simulink model "ATOM_parking_chain"  (R2026a)
settings: Solver=ode4  StopTime=100  FixedStep=0.01
StopFcn:
  | % Put every new figure in the same MATLAB Figures window as a docked tab.
  | set(groot, 'defaultFigureWindowStyle', 'docked');
  | 
  | if exist('costmap_active', 'var') && ...
  |         exist('vehicle', 'var') && ...
  |         exist('parking_path', 'var') && ...
  |         ~isempty(parking_path)
  | 
  |     plotPlan(costmap_active, vehicle, parking_path);
  | 
  | else
  | 
  |     warning('No valid parking path is available for plotting.');
  | 
  | end
  | 
  | PlotControllerReferences( ...
  |     out.controller_reference_log);
  | 
  | PlotControllerTracking( ...
  |     out.controller_tracking_log);
undefined symbols (not defined in the file): lateral, longitudinal, stanley, vehicle
(part 10 of 11)

== matlab function ATOM_parking_chain/Plot vehicle1/Plot Vehicle Rear reference frame ==
  settings: updateMethod=DISCRETE
  data: kinematic input Bus: KinematicStateBus; steer_front input double; steer_rear input double; veh input; traj input; costmap input
   function plotVehicleRear(kinematic, steer_front, steer_rear, veh, traj, costmap)
  coder.extrinsic('imagesc','colormap','evalin');
%% Vehicle parameters

L  = veh(3);
track = veh(4);

front_overhang = veh(5);
rear_overhang  = veh(6);
left_overhang = veh(7);
right_overhang = veh(8);

vehicle_length  = L + front_overhang + rear_overhang;
vehicle_width = track + left_overhang + right_overhang;

wheel_width = veh(2);
wheel_radius = veh(1);

%% Reference trajectory

x_ref = evalin('base', 'parking_path(:,1)');
y_ref = evalin('base', 'parking_path(:,2)');


%% Current kinematic state

x = kinematic.pose.position.x;
y = kinematic.pose.position.y;

qz = kinematic.pose.orientation.z;
qw = kinematic.pose.orientation.w;

yaw = 2*atan2(qz,qw);

vx = kinematic.twist.linear.x;

steer_front = steer_front;
steer_rear = steer_rear;

%% Position and orientation vehicle body

vehicle_body = [L+front_overhang vehicle_width/2;
                L+front_overhang -vehicle_width/2;
                -rear_overhang -vehicle_width/2;
                -rear_overhang vehicle_width/2;
                L+front_overhang vehicle_width/2];

R_body = [ cos(yaw) -sin(yaw)
    sin(yaw)  cos(yaw) ];

body_world = (R_body*vehicle_body')';

body_world(:,1)=body_world(:,1)+x;
body_world(:,2)=body_world(:,2)+y;


%% Position and orientation wheels

wheel_body = [wheel_radius  wheel_width/2
                wheel_radius -wheel_width/2
                -wheel_radius -wheel_width/2
                -wheel_radius  wheel_width/2
                wheel_radius  wheel_width/2];

FL = [L  track/2];
FR = [L -track/2];
RL = [0  track/2];
RR = [0 -track/2];

centers = [FL;
    FR;
    RL;
    RR];

centers = (R_body*centers')';

centers(:,1) = centers(:,1)+x;
centers(:,2) = centers(:,2)+y;

wheelFL = transformWheel(centers(1,:),steer_front,yaw,wheel_body);
wheelFR = transformWheel(centers(2,:),steer_front,yaw,wheel_body);
wheelRL = transformWheel(centers(3,:),steer_rear,yaw,wheel_body);
wheelRR = transformWheel(centers(4,:),steer_rear,yaw,wheel_body);



persistent hFig
persistent ax
persistent hBody
persistent hWheelFL
persistent hWheelFR
persistent hWheelRL
persistent hWheelRR
persistent hTrajectory
persistent TrajX
persistent TrajY
persistent hRefTraj 


if isempty(hBody)
    hFig = figure(20);
    clf

    ax = axes(hFig);

    hold(ax,'on')
    axis(ax,'equal')
    grid(ax,'on')


    xlabel(ax,'x [m]')
    ylabel(ax,'y [m]')

    % --- obstacles: the same costmap the planner used ---
    res = double(costmap.info.resolution);
    W   = double(costmap.info.width);
    H   = double(costmap.info.height);
    ox  = double(costmap.info.origin.position.x);
    oy  = double(costmap.info.origin.position.y);
    g   = double(costmap.data);
    imagesc(ax, ox+(0:W-1)*res, oy+(0:H-1)*res, g, 'AlphaData', (g>=100)*0.55);
    colormap(ax, [1 1 1; 0.85 0.25 0.25]);
    set(ax, 'YDir','normal', 'Layer','top');

    hBody = plot(body_world(:,1),...
        body_world(:,2),...
        'k','LineWidth',2);

    hWheelFL = plot(wheelFL(:,1),...
        wheelFL(:,2),...
        'r','LineWidth',2);

    hWheelFR = plot(wheelFR(:,1),...
        wheelFR(:,2),...
        'r','LineWidth',2);

    hWheelRL = plot(wheelRL(:,1),...
        wheelRL(:,2),...
        'b','LineWidth',2);

    hWheelRR = plot(wheelRR(:,1),...
        wheelRR(:,2),...
        'b','LineWidth',2);

    TrajX = x;
    TrajY = y;

   hTrajectory = plot(TrajX, TrajY, 'g', 'LineWidth', 3);
   hRefTraj    = plot(x_ref, y_ref, 'b', 'LineWidth', 1);

else

    set(hBody,...
        'XData',body_world(:,1),...
        'YData',body_world(:,2));

    set(hWheelFL,...
        'XData',wheelFL(:,1),...
        'YData',wheelFL(:,2));

    set(hWheelFR,...
        'XData',wheelFR(:,1),...
        'YData',wheelFR(:,2));

    set(hWheelRL,...
        'XData',wheelRL(:,1),...
        'YData',wheelRL(:,2));

    set(hWheelRR,...
        'XData',wheelRR(:,1),...
        'YData',wheelRR(:,2));

    TrajX(end+1) = x;
    TrajY(end+1) = y;

 
    set(hTrajectory,...
        'XData',TrajX,...
        'YData',TrajY);

    set(hRefTraj,...
        'XData',x_ref,...
        'YData',y_ref);

end

   xlim(ax, [-16 16])
   ylim(ax, [-14 14])

% xlim([-20 20])
% ylim([-20 20])

drawnow limitrate


end

== matlab function ATOM_parking_chain/Plot vehicle1/Plot vehicle Front reference frame ==
  settings: updateMethod=DISCRETE
  data: kinematic input Bus: KinematicStateBus; steer_front input double; steer_rear input double; veh input; traj input
function plotVehicleFront(kinematic, steer_front, steer_rear, veh, traj)

%% Vehicle parameters

L  = veh(3);
track = veh(4);

front_overhang = veh(5);
rear_overhang  = veh(6);
left_overhang = veh(7);
right_overhang = veh(8);

vehicle_length  = L + front_overhang + rear_overhang;
vehicle_width = track + left_overhang + right_overhang;

wheel_width = veh(2);
wheel_radius = veh(1);

%% Reference trajectory

x_ref = traj.pose.position.x;
y_ref = traj.pose.position.y;

yaw_ref = zeros(length(x_ref),1);


for i=1:length(x_ref)

    yaw_ref(i)=2*atan2(...
        traj.pose.orientation.qz(i),...
        traj.pose.orientation.qw(i));
end


%% Current kinematic state

x = kinematic.pose.position.x;
y = kinematic.pose.position.y;

qz = kinematic.pose.orientation.z;
qw = kinematic.pose.orientation.w;

yaw = 2*atan2(qz,qw);

vx = kinematic.twist.linear.x;

steer_front = steer_front;
steer_rear = steer_rear;

%% Position and orientation vehicle body

vehicle_body = [front_overhang vehicle_width/2;
                front_overhang -vehicle_width/2;
                -L-rear_overhang -vehicle_width/2;
                -L-rear_overhang vehicle_width/2;
                front_overhang vehicle_width/2];

R_body = [ cos(yaw) -sin(yaw)
    sin(yaw)  cos(yaw) ];

body_world = (R_body*vehicle_body')';

body_world(:,1)=body_world(:,1)+x;
body_world(:,2)=body_world(:,2)+y;


%% Position and orientation wheels

wheel_body = [wheel_radius  wheel_width/2
                wheel_radius -wheel_width/2
                -wheel_radius -wheel_width/2
                -wheel_radius  wheel_width/2
                wheel_radius  wheel_width/2];

FL = [0  track/2];
FR = [0 -track/2];
RL = [-L  track/2];
RR = [-L -track/2];

centers = [FL;
    FR;
    RL;
    RR];

centers = (R_body*centers')';

centers(:,1) = centers(:,1)+x;
centers(:,2) = centers(:,2)+y;

wheelFL = transformWheel(centers(1,:),steer_front,yaw,wheel_body);
wheelFR = transformWheel(centers(2,:),steer_front,yaw,wheel_body);
wheelRL = transformWheel(centers(3,:),steer_rear,yaw,wheel_body);
wheelRR = transformWheel(centers(4,:),steer_rear,yaw,wheel_body);



persistent hFig
persistent ax
persistent hBody
persistent hWheelFL
persistent hWheelFR
persistent hWheelRL
persistent hWheelRR
persistent hTrajectory
persistent TrajX
persistent TrajY
persistent hRefTraj 
persistent hArrow


if isempty(hBody)
    hFig = figure(13);
    clf

    ax = axes(hFig);

    hold(ax,'on')
    axis(ax,'equal')
    grid(ax,'on')


    xlabel(ax,'x [m]')
    ylabel(ax,'y [m]')

    hBody = plot(body_world(:,1),...
        body_world(:,2),...
        'k','LineWidth',2);

    hWheelFL = plot(wheelFL(:,1),...
        wheelFL(:,2),...
        'r','LineWidth',2);

    hWheelFR = plot(wheelFR(:,1),...
        wheelFR(:,2),...
        'r','LineWidth',2);

    hWheelRL = plot(wheelRL(:,1),...
        wheelRL(:,2),...
        'b','LineWidth',2);

    hWheelRR = plot(wheelRR(:,1),...
        wheelRR(:,2),...
        'b','LineWidth',2);

    TrajX = x;
    TrajY = y;

    hTrajectory = plot(TrajX,...
                       TrajY,...
                       'g','LineWidth',1);

    hRefTraj=plot(x_ref,y_ref,'b','LineWidth',2);

    step=5;

    hArrow=quiver(...
        x_ref(1:step:end),...
        y_ref(1:step:end),...
        cos(yaw_ref(1:step:end)),...
        sin(yaw_ref(1:step:end)),...
        0.5,...
        'r');

else

    set(hBody,...
        'XData',body_world(:,1),...
        'YData',body_world(:,2));

    set(hWheelFL,...
        'XData',wheelFL(:,1),...
        'YData',wheelFL(:,2));

    set(hWheelFR,...
        'XData',wheelFR(:,1),...
        'YData',wheelFR(:,2));

    set(hWheelRL,...
        'XData',wheelRL(:,1),...
        'YData',wheelRL(:,2));

    set(hWheelRR,...
        'XData',wheelRR(:,1),...
        'YData',wheelRR(:,2));

    TrajX(end+1) = x;
    TrajY(end+1) = y;

 
    set(hTrajectory,...
        'XData',TrajX,...
        'YData',TrajY);

    set(hRefTraj,...
        'XData',x_ref,...
        'YData',y_ref);

    

end

margin = 12;
xlim(ax, [x-margin x+margin])
ylim(ax, [y-margin y+margin])

% xlim([-20 20])
% ylim([-20 20])

drawnow limitrate


end

== matlab function ATOM_parking_chain/Plot vehicle1/RearToFrontOdometry ==
  data: rear_pose input Bus: KinematicStateBus; front_pose output Bus: KinematicStateBus; wheel_base input
function front_pose = RearToFrontOdometry( ...
    rear_pose,...
    wheel_base)


front_pose = rear_pose;


qx = rear_pose.pose.orientation.x;
qy = rear_pose.pose.orientation.y;
qz = rear_pose.pose.orientation.z;
qw = rear_pose.pose.orientation.w;


yaw = QuaternionToYaw(qx,qy,qz,qw);



front_pose.pose.position.x = ...
    rear_pose.pose.position.x + ...
    wheel_base*cos(yaw);


front_pose.pose.position.y = ...
    rear_pose.pose.position.y + ...
    wheel_base*sin(yaw);


front_pose.pose.position.z = ...
    rear_pose.pose.position.z;



% orientation unchanged

front_pose.pose.orientation = ...
    rear_pose.pose.orientation;


% Linear velocity referred to front axle

front_pose.twist.linear.x = rear_pose.twist.linear.x ...
    - rear_pose.twist.angular.z ...
    * wheel_base*sin(yaw);


front_pose.twist.linear.y = rear_pose.twist.linear.y ...
    + rear_pose.twist.angular.z ...
    * wheel_base*cos(yaw);


front_pose.twist.linear.z = rear_pose.twist.linear.z;


end

== matlab function ATOM_parking_chain/Parking Scenario/Costmap generation: perpendicular lot/Perpendicular Parking ==
  settings: updateMethod=DISCRETE
  data: veh input; costmap output Bus: OccupancyGridBus; start_pose output; goal_pose output
function [costmap, start_pose, goal_pose] = costmapPerpendicularLot(veh)
%COSTMAPPERPENDICULARLOT  Single row of 7 bays, one left empty at x = 0.
%
% Reproduces autoware_costmap_generator geometry:
%   grid_resolution 0.3, grid_length_x/y 70.0, expand_polygon_size 0.5
% The primitives layer is INVERTED: background occupied, lot carved out.

persistent occ

res = 0.3;   W = 234;   H = 234;
origin_x = -(W/2)*res;
origin_y = -(H/2)*res;

bay_x     = (-3:3)*3.6;      % 7 bays, 3.6 m pitch
bay_y     = 8.75;
empty_bay = 4;               % x = 0

if isempty(occ)
    [IX, IY] = meshgrid(0:W-1, 0:H-1);
    X = origin_x + IX*res;
    Y = origin_y + IY*res;

    lot_x = [-15  15  15 -15];
    lot_y = [-12 -12  12  12];
    occ = ones(H,W);
    occ(inpolygon(X, Y, lot_x, lot_y)) = 0;

    car_len = veh(5) + veh(3) + veh(6);
    car_wid = veh(4) + veh(7) + veh(8);
    expand  = 0.5;
    L = car_len + expand;
    D = car_wid + expand;

    for k = 1:7
        if k ~= empty_bay
            qx = [ D/2 -D/2 -D/2  D/2] + bay_x(k);
            qy = [ L/2  L/2 -L/2 -L/2] + bay_y;
            occ(inpolygon(X, Y, qx, qy)) = 1;
        end
    end
end

start_pose = [0, 0,    0];
goal_pose  = [0, 7.75, pi/2];

costmap.info.resolution           = res;
costmap.info.width                = uint32(W);
costmap.info.height               = uint32(H);
costmap.info.origin.position.x    = origin_x;
costmap.info.origin.position.y    = origin_y;
costmap.info.origin.position.z    = 0;
costmap.info.origin.orientation.x = 0;
costmap.info.origin.orientation.y = 0;
costmap.info.origin.orientation.z = 0;
costmap.info.origin.orientation.w = 1;
costmap.data                      = int8(occ*100);
end

== matlab function ATOM_parking_chain/Plot vehicle1/SetStanleyTrajectory/Resample Trajectory ==
  data: trajectory_in input Bus: TrajectoryDataBus; trajectory_out output Bus: TrajectoryDataBus; resample_interval_dist input; nearest_seg_idx input; ego_offset_to_segment input
function trajectory_out = resampleTrajectoryByDistance( ...
    trajectory_in, ...
    resample_interval_dist, ...
    nearest_seg_idx, ...
    ego_offset_to_segment)


%% ============================================================
% RESAMPLE TRAJECTORY BY ARC LENGTH
%
% Equivalent to:
%
% MPCUtils::resampleMPCTrajectoryByDistance()
%
% Adapted for Stanley controller.
%
% Unlike MPC:
% - no MPCTrajectory conversion
% - no curvature resampling
% - no optimization variables
%
% The trajectory is directly interpolated in arc length.
%
% ATTENTION:
% 
% Resampling is not actuated in Simulink since in/out buses present fixed sizes.
% See NOTE at the end of this function.
%
% =============================================================


% N = length(trajectory_in.pose.position.x);
% 
% 
% if N < 2
% 
%     trajectory_out = trajectory_in;
%     return
% 
% end
% 
% 
% 
% %% ============================================================
% % Compute arc length
% % =============================================================
% 
% x = trajectory_in.pose.position.x;
% y = trajectory_in.pose.position.y;
% 
% 
% arc_length = zeros(N,1);
% 
% 
% for i = 2:N
% 
%     dx = x(i)-x(i-1);
%     dy = y(i)-y(i-1);
% 
%     arc_length(i)= ...
%         arc_length(i-1)+sqrt(dx^2+dy^2);
% 
% end
% 
% 
% 
% if isempty(arc_length)
% 
%     trajectory_out = trajectory_in;
%     return
% 
% end
% 
% 
% 
% %% ============================================================
% % Ego position along trajectory
% %
% % Equivalent to:
% %
% % input_arclength(nearest_seg_idx)
% % + ego_offset_to_segment
% %
% % =============================================================
% 
% 
% ego_s = arc_length(nearest_seg_idx) ...
%         + ego_offset_to_segment;
% 
% 
% ego_s = min(max(ego_s,0),arc_length(end));
% 
% 
% 
% %% ============================================================
% % Generate resampling points
% %
% % Same strategy as Autoware:
% % - backward from ego
% % - forward from ego
% %
% % =============================================================
% 
% 
% output_s = [];
% 
% 
% % backward direction
% 
% s = ego_s;
% 
% while s >= 0
% 
%     output_s = [s output_s]; %#ok<AGROW>
% 
%     s = s - resample_interval_dist;
% 
% end
% 
% 
% 
% % forward direction
% 
% s = ego_s + resample_interval_dist;
% 
% 
% while s < arc_length(end)
% 
%     output_s(end+1)=s; % #ok<AGROW>
% 
%     s = s + resample_interval_dist;
% 
% end
% 
% 
% 
% %% ============================================================
% % Interpolation
% % =============================================================
% 
% 
% x_new = interp1( ...
%     arc_length,...
%     x,...
%     output_s,...
%     'linear');
% 
% 
% 
% y_new = interp1( ...
%     arc_length,...
%     y,...
%     output_s,...
%     'linear');
% 
% 
% 
% z = trajectory_in.pose.position.z;
% 
% z_new = interp1( ...
%     arc_length,...
%     z,...
%     output_s,...
%     'linear');
% 
% 
% 
% %% ============================================================
% % Quaternion / yaw interpolation
% %
% % Stanley works with yaw.
% % Therefore interpolate yaw and rebuild quaternion.
% %
% % =============================================================
% 
% 
% yaw = QuaternionToYaw( ...
%     trajectory_in.pose.orientation.qx,...
%     trajectory_in.pose.orientation.qy,...
%     trajectory_in.pose.orientation.qz,...
%     trajectory_in.pose.orientation.qw);
% 
% 
% 
% % avoid discontinuity
% 
% yaw = unwrap(yaw);
% 
% 
% 
% yaw_new = interp1( ...
%     arc_length,...
%     yaw,...
%     output_s,...
%     'linear');
% 
% 
% 
% %% ============================================================
% % Velocity interpolation
% %
% % Autoware uses linear interpolation
% % =============================================================
% 
% 
% vel_new = interp1( ...
%     arc_length,...
%     trajectory_in.longitudinal_velocity_mps,...
%     output_s,...
%     'linear');
% 
% 
% 
% lat_vel_new = interp1( ...
%     arc_length,...
%     trajectory_in.lateral_velocity_mps,...
%     output_s,...
%     'linear');
% 
% 
% 
% acc_new = interp1( ...
%     arc_length,...
%     trajectory_in.acceleration_mps2,...
%     output_s,...
%     'linear');
% 
% 
% 
% %% ============================================================
% % Build output structure
% % =============================================================
% 
% 
% M = length(output_s);
% 
% 
% trajectory_out.pose.position.x = x_new;
% trajectory_out.pose.position.y = y_new;
% trajectory_out.pose.position.z = z_new;
% 
% 
% 
% [qx,qy,qz,qw] = yawToQuaternion(yaw_new);
% 
% 
% 
% trajectory_out.pose.orientation.qx = qx;
% trajectory_out.pose.orientation.qy = qy;
% trajectory_out.pose.orientation.qz = qz;
% trajectory_out.pose.orientation.qw = qw;
% 
% 
% 
% trajectory_out.longitudinal_velocity_mps = vel_new;
% 
% trajectory_out.lateral_velocity_mps = lat_vel_new;
% 
% trajectory_out.acceleration_mps2 = acc_new;
% 
% 
% 
% % steering values are kept
% 
% trajectory_out.front_wheel_angle_rad = ...
%     interp1( ...
%     arc_length,...
%     trajectory_in.front_wheel_angle_rad,...
%     output_s,...
%     'linear');
% 
% 
% trajectory_out.rear_wheel_angle_rad = ...
%     interp1( ...
%     arc_length,...
%     trajectory_in.rear_wheel_angle_rad,...
%     output_s,...
%     'linear');
% 
% 


%% ============================================================
% NOTE (Simulink Implementation)
%
% The trajectory resampling algorithm reported above is equivalent
% to the implementation adopted by Autoware.
%
% However, the main objective of the present work is the development
% and validation of the 4WS Stanley Controller rather than the
% trajectory preprocessing module.
%
% Since Simulink requires fixed-size bus signals, the resampled
% trajectory is not generated in the simulation model.
%
% The original input trajectory is therefore directly propagated to
% the controller, preserving its fixed dimension and avoiding the
% introduction of variable-length signals.
%
% Consequently, the following assignment overwrites the resampled
% trajectory computed above.
%
% ============================================================

trajectory_out = trajectory_in;

end

== matlab function ATOM_parking_chain/Plot vehicle1/SetStanleyTrajectory/calcLongOffsetToSegment ==
  data: seg_idx input; ego_pose input; trajectory input Bus: TrajectoryDataBus; ego_offset_to_segment output
function ego_offset_to_segment = calcLongOffsetToSegment(seg_idx, ego_pose, trajectory)

ego_offset_to_segment = calcLongitudinalOffsetToSegment(trajectory, seg_idx, ego_pose);

end

== matlab function ATOM_parking_chain/Plot vehicle1/SetStanleyTrajectory/findFirstNearestSegmentIndexWithSoftConstraints ==
  data: trajectory input; dist_threshold input; yaw_threshold input; nearest_seg_idx output; pose input
function nearest_seg_idx = findNearestSegmentIndexWithSoftConstraints( ...
    trajectory, dist_threshold, yaw_threshold, pose)


%% Step 1:
% Find nearest point index

nearest_idx = findFirstNearestIndexWithSoftConstraints( ...
    trajectory, ...
    pose, ...
    dist_threshold, ...
    yaw_threshold);


N = length(trajectory.pose.position.x);


%% Step 2:
% Convert point index into segment index

% First point
if nearest_idx == 1

    nearest_seg_idx = 1;
    return

end


% Last point
if nearest_idx == N

    nearest_seg_idx = N-1;
    return

end



%% Step 3:
% Determine whether ego lies before or after nearest point
%
% Equivalent to Autoware:
%
% signed_length =
% calcLongitudinalOffsetToSegment(points,
%                                 nearest_idx,
%                                 pose.position)


signed_length = calcLongitudinalOffsetToSegment( ...
    trajectory,...
    nearest_idx,...
    pose);



%% Step 4:
% Choose segment

if signed_length <= 0

    % ego is before nearest point
    %
    % Autoware:
    % return nearest_idx - 1;

    nearest_seg_idx = nearest_idx - 1;


else

    % ego is after nearest point
    %
    % Autoware:
    % return nearest_idx;

    nearest_seg_idx = nearest_idx;

end


end

== matlab function ATOM_parking_chain/Parking Scenario/MATLAB Function ==
  data: segment_done input; segment_request output; segment_count input; maneuver_complete output
function [segment_request, maneuver_complete] = ...
    segmentManager(segment_done, segment_count)
%SEGMENTMANAGER
% Advance exactly once when the current segment is completed.

persistent active_segment previous_done complete_latched

if isempty(active_segment)
    active_segment  = 1.0;
    previous_done   = false;
    complete_latched = false;
end

% Convert the inputs into known scalar types.
done_now = logical(segment_done);
count = max(0.0, floor(double(segment_count)));

% Protect against an active index larger than the available count.
if count > 0 && active_segment > count
    active_segment = count;
end

% Detect only the transition from not-done to done.
done_rising_edge = done_now && ~previous_done;

if done_rising_edge && count > 0

    if active_segment < count

        % Another segment exists.
        active_segment = active_segment + 1.0;

    else

        % The final segment has been completed.
        complete_latched = true;

    end
end

previous_done = done_now;

segment_request  = active_segment;
maneuver_complete = complete_latched;
end

== matlab function ATOM_parking_chain/parking_velocity_smoother/MATLAB Function ==
  data: trajectory_in input Bus: TrajectoryDataBus size=1; trajectory_out output Bus: TrajectoryDataBus size=1
function trajectory_out = parkingVelocitySmoother(trajectory_in)
%#codegen
%
% Generate the longitudinal velocity and acceleration reference
% for one forward or reverse parking segment.

% Preserve all fields of the original trajectory bus.
trajectory_out = trajectory_in;

% The parking trajectory contains exactly 100 points.
N = 100;

%% 1. Velocity-profile parameters

% v_max       = 0.30; %0.50;   % previously 1.00  % desired maximum parking speed [m/s]
% a_accel_max = 0.25; %0.5;   % previously 1.00   % from velocity_smoother.max_acc

v_max           = 0.80;
v_curve         = 0.30;
steer_threshold = 0.10;

a_accel_max = 0.25;
a_decel_max = 0.50;

% Existing lateral-acceleration limit from velocity_smoother_params.m.
a_lat_max = 1.00;     % maximum lateral acceleration [m/s^2]

% Existing curvature-calculation distance from
% velocity_smoother_params.m.
curvature_calculation_distance = 2.00;   % [m]

%% 2. Read the trajectory data

px = trajectory_in.pose.position.x;
py = trajectory_in.pose.position.y;

% rear_angle = trajectory_in.rear_wheel_angle_rad;

front_angle = trajectory_in.front_wheel_angle_rad;
rear_angle  = trajectory_in.rear_wheel_angle_rad;


% At this stage, the incoming velocity is used only to determine
% whether the segment is forward or reverse.
raw_velocity = trajectory_in.longitudinal_velocity_mps;

%% 3. Determine the segment direction

% Default to forward if no nonzero direction can be found.
gear = 1.0;

for k = 1:N
    if abs(raw_velocity(k)) > 1e-6
        gear = sign(raw_velocity(k));
        break;
    end
end

%% 4. Calculate distance between consecutive trajectory points

ds = zeros(N-1,1);
path_length = 0.0;

for k = 1:N-1
    dx = px(k+1) - px(k);
    dy = py(k+1) - py(k);

    ds(k) = hypot(dx,dy);
    path_length = path_length + ds(k);
end

% Use higher speed only when the active segment is long enough.
% long_segment_threshold = 2.0;   % [m]

% if path_length > long_segment_threshold
%     v_max       = 0.80;   % [m/s]
%     a_accel_max = 0.50;   % [m/s^2]
% end

%% 5. Calculate trajectory curvature

% pathToTrajectory resamples the segment at approximately equal
% distances, so an index separation can represent the requested
% curvature-calculation distance.

point_interval = path_length / (N-1);

idx_dist = 1;

if point_interval > 1e-6
    idx_dist = floor( ...
        curvature_calculation_distance / point_interval);
end

% Three curvature points must remain inside the trajectory.
max_idx_dist = floor((N-1)/2);

idx_dist = max(1,min(idx_dist,max_idx_dist));

curvature = zeros(N,1);

for k = 2:N-1

    idx_prev = k - min(idx_dist,k-1);
    idx_next = k + min(idx_dist,N-k);

    x1 = px(idx_prev);
    y1 = py(idx_prev);

    x2 = px(k);
    y2 = py(k);

    x3 = px(idx_next);
    y3 = py(idx_next);

    d12 = hypot(x2-x1,y2-y1);
    d23 = hypot(x3-x2,y3-y2);
    d31 = hypot(x1-x3,y1-y3);

    denominator = d12*d23*d31;

    if abs(denominator) > 1e-10

        curvature(k) = 2.0 * ( ...
            (x2-x1)*(y3-y1) - ...
            (y2-y1)*(x3-x1)) / denominator;

    else

        % Degenerate or repeated trajectory points.
        curvature(k) = 0.0;

    end
end

% Complete the two boundary values.
curvature(1) = curvature(2);
curvature(N) = curvature(N-1);

%% 6. Build the speed ceiling

% Begin with the requested maximum parking speed.
speed_limit = v_max * ones(N,1);

% Slow down whenever the planned wheels are steering.
for k = 1:N

    steering_activity = max( ...
        abs(front_angle(k)), ...
        abs(rear_angle(k)));

    if steering_activity > steer_threshold
        speed_limit(k) = min(speed_limit(k),v_curve);
    end
end


% Reduce the speed wherever the trajectory curvature would cause the
% lateral acceleration to exceed a_lat_max.
%
% Current 4WS model relation:
%
%     a_lat = vx^2 * curvature / cos(delta_r)
%
% Therefore:
%
%     vx_max = sqrt(a_lat_max*cos(delta_r)/abs(curvature))

for k = 1:N

    kappa = abs(curvature(k));

    if kappa > 1e-6

        cos_rear = cos(rear_angle(k));

        % Numerical protection. With the present steering limits,
        % cos(rear_angle) should remain positive.
        if cos_rear < 1e-6
            cos_rear = 1e-6;
        end

        v_lateral_max = sqrt( ...
            a_lat_max*cos_rear/kappa);

        % The final local ceiling is the smaller of:
        %   1. the 2 m/s parking limit;
        %   2. the curvature-based lateral limit.
        speed_limit(k) = min( ...
            speed_limit(k), ...
            v_lateral_max);
    end
end

%% 7. Backward pass: ensure that the vehicle can stop

speed_backward = speed_limit;

% Every parking segment ends at rest.
speed_backward(N) = 0.0;

for k = N-1:-1:1

    % Maximum speed at point k from which the vehicle can still
    % brake to speed_backward(k+1).
    reachable_speed = sqrt( ...
        speed_backward(k+1)^2 + ...
        2.0*a_decel_max*ds(k));

    speed_backward(k) = min( ...
        speed_backward(k), ...
        reachable_speed);
end

%% 8. Forward pass: enforce the acceleration limit

speed_magnitude = speed_backward;

% Every segment starts at rest, including after a gear reversal.
speed_magnitude(1) = 0.0;

for k = 2:N

    % Maximum speed reachable from the previous point without
    % exceeding a_accel_max.
    reachable_speed = sqrt( ...
        speed_magnitude(k-1)^2 + ...
        2.0*a_accel_max*ds(k-1));

    speed_magnitude(k) = min( ...
        speed_backward(k), ...
        reachable_speed);
end

%% 9. Calculate the compatible acceleration reference

acceleration_magnitude = zeros(N,1);

for k = 1:N-1

    if ds(k) > 1e-6

        acceleration_magnitude(k) = ...
            (speed_magnitude(k+1)^2 - ...
             speed_magnitude(k)^2) / ...
            (2.0*ds(k));

    else

        % Protect against duplicate consecutive points.
        acceleration_magnitude(k) = 0.0;

    end
end

% The vehicle remains stopped at the segment endpoint.
acceleration_magnitude(N) = 0.0;

%% 10. Apply the forward or reverse sign

trajectory_out.longitudinal_velocity_mps = ...
    gear*speed_magnitude;

trajectory_out.acceleration_mps2 = ...
    gear*acceleration_magnitude;

end

== matlab function ATOM_parking_chain/Subsystem/parkingLongitudinalController ==
  data: tx input; a_cmd output; ty input; tvx input; tax input; s_now input; vx input; longitudinal_mode input; a_ref_out output; v_ref_out output
function [a_cmd,a_ref_out,v_ref_out] = parkingLongitudinalController( ...
    tx, ty, tvx, tax, s_now, vx, longitudinal_mode)
%#codegen
%
% Independent longitudinal parking controller.
%
% Inputs:
%   tx, ty  : trajectory position arrays
%   tvx     : signed velocity reference array
%   tax     : signed acceleration feedforward array
%   s_now   : current progress along the trajectory
%   vx      : measured longitudinal velocity
%   longitudinal_mode:
%             0 = normal profile tracking
%             1 = terminal creep
%             2 = stop
%
% Output:
%   a_cmd   : commanded longitudinal acceleration

N = 100;

% Normal velocity-tracking gain.
Kp = 1.0;

% Stronger gain used only when stopping at a segment endpoint.
% With the 1 m/s^2 command limit, this requests maximum braking whenever
% the speed magnitude is greater than or equal to 0.20 m/s.
Kp_stop = 5.0;

% Existing velocity-smoother longitudinal acceleration limit.
a_cmd_limit = 1.0;

terminal_creep_speed = 0.05;

%% Construct trajectory arc length

s = zeros(N,1);

for k = 2:N
    s(k) = s(k-1) + hypot( ...
        tx(k)-tx(k-1), ...
        ty(k)-ty(k-1));
end

%% Read the feedforward references at the current progress

v_ref = lookupS(s,tvx,s_now);
a_ref = lookupS(s,tax,s_now);

%% Determine the forward or reverse direction

gear = 1.0;

for k = 1:N
    if abs(tvx(k)) > 1e-6
        gear = sign(tvx(k));
        break;
    end
end

%% Apply the maneuver-supervisor mode
%% Apply the maneuver-supervisor mode

% Use the normal tracking gain unless stop mode selects the stronger gain.
Kp_active = Kp;

if longitudinal_mode == 2.0

    % Stop mode.
    % Drive the measured velocity firmly toward zero.
    v_ref = 0.0;
    a_ref = 0.0;
    Kp_active = Kp_stop;

elseif longitudinal_mode == 1.0

    % Very slow endpoint correction.
    v_ref = gear*terminal_creep_speed;
    a_ref = 0.0;

end

% Acceleration reference currently selected at the vehicle's progress.
a_ref_out = a_ref;
v_ref_out = v_ref;
%% Feedforward plus velocity-error correction

%% Feedforward plus velocity-error correction

speed_error = v_ref - vx;

% Express the measured and reference velocities in the direction of the
% current segment. Positive means movement in the intended gear direction.
speed_in_gear = gear * vx;
reference_speed_in_gear = gear * v_ref;
feedforward_in_gear = gear * a_ref;

% A negative feedforward value means braking.
%
% Apply braking feedforward only while the vehicle is moving faster than
% its reference. Once the vehicle is at or below the reference speed,
% remove the braking feedforward and let the velocity feedback correct it.
%
% This also prevents the controller from intentionally accelerating the
% vehicle in the opposite direction before the segment manager authorizes
% a gear change.
a_feedforward = a_ref;

if feedforward_in_gear < 0.0 && ...
        speed_in_gear <= reference_speed_in_gear

    a_feedforward = 0.0;

end

a_unsaturated = ...
    a_feedforward + Kp_active*speed_error;

a_cmd = max( ...
    -a_cmd_limit, ...
    min(a_cmd_limit,a_unsaturated));

end

%--------------------------------------------------------------------------
function value = lookupS(sv,vv,s_query)
% Linear interpolation of a trajectory quantity by path distance.

n = numel(sv);
value = vv(n);

if s_query <= sv(1)
    value = vv(1);
    return;
end

if s_query >= sv(n)
    return;
end

for k = 1:n-1

    if s_query <= sv(k+1)

        ds = sv(k+1)-sv(k);

        if ds < 1e-12
            value = vv(k+1);
        else
            ratio = (s_query-sv(k))/ds;
            value = vv(k) + ratio*(vv(k+1)-vv(k));
        end

        return;
    end
end

end

== matlab function ATOM_parking_chain/Parking Scenario/Costmap generation: obstacle1/MATLAB Function ==
  settings: updateMethod=DISCRETE
  data: costmap output Bus: OccupancyGridBus; start_pose output; goal_pose output; veh input
function [costmap, start_pose, goal_pose] = costmapOffsetDock(veh)
%COSTMAPOFFSETDOCK  A short, angled parking bay beside a narrow aisle.
% Paste into a duplicate of an existing costmap MATLAB Function block.
% Inputs/outputs and the 234-by-234 int8 payload match the current model.
% Poses refer to the rear-axle centre; headings are in radians.

%% Map and scene dimensions [m]
res = 0.20;
W = 234;
H = 234;
origin_x = -(W/2)*res;
origin_y = -(H/2)*res;

aisle_width = 3.20;
aisle_x_min = -8.9;
aisle_x_max =  7.1;
aisle_center_y = 0.10;

bay_length = 4.30;
bay_width  = 3.40;
bay_angle  = 15*pi/180;
bay_center_x = 0.0;
bay_center_y = 2.70;

%% Rear-axle start and goal poses
start_pose = [-5.0, 0.0, pi];

% The bay centre is a BODY-centre position, not a rear-axle position.
body_center_from_rear_axle = (veh(3) + veh(5) - veh(6))/2;
goal_pose = [ ...
    bay_center_x - body_center_from_rear_axle*cos(bay_angle), ...
    bay_center_y - body_center_from_rear_axle*sin(bay_angle), ...
    bay_angle];

%% Occupancy grid
% Stateless: each call reflects the dimensions above, without a cached map.
[IX,IY] = meshgrid(0:W-1,0:H-1);
X = origin_x + IX*res;
Y = origin_y + IY*res;

% Avoid asymmetric inclusion of boundary points due to floating-point error.
tol = 1e-9;
% These walls coincide with cell edges. Include only complete free cells.
% The start is 0.10 m below the aisle centreline.
aisle = X >= aisle_x_min+res/2-tol & X <= aisle_x_max-res/2+tol & ...
        abs(Y-aisle_center_y) <= aisle_width/2-res/2+tol;

% Coordinates along/across the angled bay.
dx = X-bay_center_x;
dy = Y-bay_center_y;
along  =  cos(bay_angle)*dx + sin(bay_angle)*dy;
across = -sin(bay_angle)*dx + cos(bay_angle)*dy;
bay = abs(along) <= bay_length/2+tol & ...
      abs(across) <= bay_width/2+tol;

% Free space is the union of the aisle and bay. Everything else is occupied.
% No obstacle inflation is added here. The planner handles its ego margin.
occupied = ~(aisle | bay);

%% Existing OccupancyGrid bus format
costmap.info.resolution = res;
costmap.info.width  = uint32(W);
costmap.info.height = uint32(H);
costmap.info.origin.position.x = origin_x;
costmap.info.origin.position.y = origin_y;
costmap.info.origin.position.z = 0;
costmap.info.origin.orientation.x = 0;
costmap.info.origin.orientation.y = 0;
costmap.info.origin.orientation.z = 0;
costmap.info.origin.orientation.w = 1;
costmap.data = int8(occupied).*int8(100);
end

== matlab function ATOM_parking_chain/Parking Scenario/Costmap generation: obstacle2/MATLAB Function ==
  settings: updateMethod=DISCRETE
  data: costmap output Bus: OccupancyGridBus; start_pose output; goal_pose output; veh input
function [costmap, start_pose, goal_pose] = costmapUndergroundParking(veh)
%COSTMAPUNDERGROUNDPARKING  Realistic reverse parking in a double-row garage.
% The target is the empty bay at x = 0 in the upper row. Parked vehicles
% surround it, an opposing row limits the aisle, and a structural column is
% located beside the entrance. Poses refer to the rear-axle centre.

%% Fixed OccupancyGrid dimensions used by the current model
res = 0.20;
W = 234;
H = 234;
origin_x = -(W/2)*res;
origin_y = -(H/2)*res;
[IX,IY] = meshgrid(0:W-1,0:H-1);
X = origin_x + IX*res;
Y = origin_y + IY*res;

%% Garage geometry [m]
aisle_width = 6.50;       % clear nominal two-way manoeuvring aisle
parking_depth = 5.20;
bay_pitch = 3.20;         % centre-to-centre bay spacing
parked_length = 4.60;     % physical parked vehicle, no inflation here
parked_width = 2.00;
pillar_size = 0.40;

garage_x_min = -11.0;
garage_x_max =  11.0;
garage_y_min = -(aisle_width/2 + parking_depth);
garage_y_max =  (aisle_width/2 + parking_depth);

% Start occupied and carve out the garage floor.
occupied = true(H,W);
garage_floor = X >= garage_x_min & X <= garage_x_max & ...
               Y >= garage_y_min & Y <= garage_y_max;
occupied(garage_floor) = false;

%% Parked vehicles
row_y = aisle_width/2 + parking_depth/2;
bay_x = (-3:3)*bay_pitch;

for k = 1:numel(bay_x)
    % Upper row: leave the centre bay empty.
    if k ~= 4
        top_car = abs(X-bay_x(k)) <= parked_width/2 & ...
                  abs(Y-row_y) <= parked_length/2;
        occupied(top_car) = true;
    end

    % Opposing row: all bays occupied.
    bottom_car = abs(X-bay_x(k)) <= parked_width/2 & ...
                 abs(Y+row_y) <= parked_length/2;
    occupied(bottom_car) = true;
end

%% Structural column beside the target bay entrance
pillar_x = bay_pitch/2;
pillar_y = aisle_width/2 + pillar_size/2 + 0.10;
pillar = abs(X-pillar_x) <= pillar_size/2 & ...
         abs(Y-pillar_y) <= pillar_size/2;
occupied(pillar) = true;

%% Parking task
% The vehicle begins beside the target bay, as it would after approaching
% through the aisle, and reverses into the upper-row space.
start_pose = [-5.0, 0.0, pi/2];
goal_pose = [0.0, row_y, -pi/2];

%% Existing OccupancyGrid bus format
costmap.info.resolution = res;
costmap.info.width = uint32(W);
costmap.info.height = uint32(H);
costmap.info.origin.position.x = origin_x;
costmap.info.origin.position.y = origin_y;
costmap.info.origin.position.z = 0;
costmap.info.origin.orientation.x = 0;
costmap.info.origin.orientation.y = 0;
costmap.info.origin.orientation.z = 0;
costmap.info.origin.orientation.w = 1;
costmap.data = int8(occupied).*int8(100);

% veh is intentionally kept as the input because the surrounding subsystem
% already supplies the 29-element vehicle vector and all costmap blocks use
% the same interface. Geometry above represents other parked vehicles.
if numel(veh) < 8
    error('costmapUndergroundParking:VehSize', ...
        'veh must be the complete vehicle-parameter vector.');
end
end

== matlab function ATOM_parking_chain/parking_velocity_smoother2/MATLAB Function ==
  data: trajectory_in input Bus: TrajectoryDataBus size=1; trajectory_out output Bus: TrajectoryDataBus size=1
function trajectory_out = parkingVelocitySmoother(trajectory_in)
%#codegen
%
% Generate the longitudinal velocity and acceleration reference
% for one forward or reverse parking segment.

% Preserve all fields of the original trajectory bus.
trajectory_out = trajectory_in;

% The parking trajectory contains exactly 100 points.
N = 100;

%% 1. Velocity-profile parameters

% v_max       = 0.30; %0.50;   % previously 1.00  % desired maximum parking speed [m/s]
% a_accel_max = 0.25; %0.5;   % previously 1.00   % from velocity_smoother.max_acc

v_max           = 0.80;
v_curve         = 0.30;
steer_threshold = 0.10;

a_accel_max = 0.25;
a_decel_max = 0.50;

% Existing lateral-acceleration limit from velocity_smoother_params.m.
a_lat_max = 1.00;     % maximum lateral acceleration [m/s^2]

% Existing curvature-calculation distance from
% velocity_smoother_params.m.
curvature_calculation_distance = 2.00;   % [m]

%% 2. Read the trajectory data

px = trajectory_in.pose.position.x;
py = trajectory_in.pose.position.y;

% rear_angle = trajectory_in.rear_wheel_angle_rad;

front_angle = trajectory_in.front_wheel_angle_rad;
rear_angle  = trajectory_in.rear_wheel_angle_rad;


% At this stage, the incoming velocity is used only to determine
% whether the segment is forward or reverse.
raw_velocity = trajectory_in.longitudinal_velocity_mps;

%% 3. Determine the segment direction

% Default to forward if no nonzero direction can be found.
gear = 1.0;

for k = 1:N
    if abs(raw_velocity(k)) > 1e-6
        gear = sign(raw_velocity(k));
        break;
    end
end

%% 4. Calculate distance between consecutive trajectory points

ds = zeros(N-1,1);
path_length = 0.0;

for k = 1:N-1
    dx = px(k+1) - px(k);
    dy = py(k+1) - py(k);

    ds(k) = hypot(dx,dy);
    path_length = path_length + ds(k);
end

% Use higher speed only when the active segment is long enough.
% long_segment_threshold = 2.0;   % [m]

% if path_length > long_segment_threshold
%     v_max       = 0.80;   % [m/s]
%     a_accel_max = 0.50;   % [m/s^2]
% end

%% 5. Calculate trajectory curvature

% pathToTrajectory resamples the segment at approximately equal
% distances, so an index separation can represent the requested
% curvature-calculation distance.

point_interval = path_length / (N-1);

idx_dist = 1;

if point_interval > 1e-6
    idx_dist = floor( ...
        curvature_calculation_distance / point_interval);
end

% Three curvature points must remain inside the trajectory.
max_idx_dist = floor((N-1)/2);

idx_dist = max(1,min(idx_dist,max_idx_dist));

curvature = zeros(N,1);

for k = 2:N-1

    idx_prev = k - min(idx_dist,k-1);
    idx_next = k + min(idx_dist,N-k);

    x1 = px(idx_prev);
    y1 = py(idx_prev);

    x2 = px(k);
    y2 = py(k);

    x3 = px(idx_next);
    y3 = py(idx_next);

    d12 = hypot(x2-x1,y2-y1);
    d23 = hypot(x3-x2,y3-y2);
    d31 = hypot(x1-x3,y1-y3);

    denominator = d12*d23*d31;

    if abs(denominator) > 1e-10

        curvature(k) = 2.0 * ( ...
            (x2-x1)*(y3-y1) - ...
            (y2-y1)*(x3-x1)) / denominator;

    else

        % Degenerate or repeated trajectory points.
        curvature(k) = 0.0;

    end
end

% Complete the two boundary values.
curvature(1) = curvature(2);
curvature(N) = curvature(N-1);

%% 6. Build the speed ceiling

% Begin with the requested maximum parking speed.
speed_limit = v_max * ones(N,1);

% Slow down whenever the planned wheels are steering.
for k = 1:N

    steering_activity = max( ...
        abs(front_angle(k)), ...
        abs(rear_angle(k)));

    if steering_activity > steer_threshold
        speed_limit(k) = min(speed_limit(k),v_curve);
    end
end


% Reduce the speed wherever the trajectory curvature would cause the
% lateral acceleration to exceed a_lat_max.
%
% Current 4WS model relation:
%
%     a_lat = vx^2 * curvature / cos(delta_r)
%
% Therefore:
%
%     vx_max = sqrt(a_lat_max*cos(delta_r)/abs(curvature))

for k = 1:N

    kappa = abs(curvature(k));

    if kappa > 1e-6

        cos_rear = cos(rear_angle(k));

        % Numerical protection. With the present steering limits,
        % cos(rear_angle) should remain positive.
        if cos_rear < 1e-6
            cos_rear = 1e-6;
        end

        v_lateral_max = sqrt( ...
            a_lat_max*cos_rear/kappa);

        % The final local ceiling is the smaller of:
        %   1. the 2 m/s parking limit;
        %   2. the curvature-based lateral limit.
        speed_limit(k) = min( ...
            speed_limit(k), ...
            v_lateral_max);
    end
end

%% 7. Backward pass: ensure that the vehicle can stop

speed_backward = speed_limit;

% Every parking segment ends at rest.
speed_backward(N) = 0.0;

for k = N-1:-1:1

    % Maximum speed at point k from which the vehicle can still
    % brake to speed_backward(k+1).
    reachable_speed = sqrt( ...
        speed_backward(k+1)^2 + ...
        2.0*a_decel_max*ds(k));

    speed_backward(k) = min( ...
        speed_backward(k), ...
        reachable_speed);
end

%% 8. Forward pass: enforce the acceleration limit

speed_magnitude = speed_backward;

% Every segment starts at rest, including after a gear reversal.
speed_magnitude(1) = 0.0;

for k = 2:N

    % Maximum speed reachable from the previous point without
    % exceeding a_accel_max.
    reachable_speed = sqrt( ...
        speed_magnitude(k-1)^2 + ...
        2.0*a_accel_max*ds(k-1));

    speed_magnitude(k) = min( ...
        speed_backward(k), ...
        reachable_speed);
end

%% 9. Calculate the compatible acceleration reference

acceleration_magnitude = zeros(N,1);

for k = 1:N-1

    if ds(k) > 1e-6

        acceleration_magnitude(k) = ...
            (speed_magnitude(k+1)^2 - ...
             speed_magnitude(k)^2) / ...
            (2.0*ds(k));

    else

        % Protect against duplicate consecutive points.
        acceleration_magnitude(k) = 0.0;

    end
end

% The vehicle remains stopped at the segment endpoint.
acceleration_magnitude(N) = 0.0;

%% 10. Apply the forward or reverse sign

trajectory_out.longitudinal_velocity_mps = ...
    gear*speed_magnitude;

trajectory_out.acceleration_mps2 = ...
    gear*acceleration_magnitude;

end

== matlab function ATOM_parking_chain/Parking Scenario1/Costmap generation: complex parking situation/MATLAB Function ==
  settings: updateMethod=DISCRETE
  data: veh input; costmap output Bus: OccupancyGridBus; start_pose output; goal_pose output
function [costmap, start_pose, goal_pose] = ...
    costmapRoadsideParallelParking(veh)
%COSTMAPROADSIDEPARALLELPARKING
% A straight road with one parallel parking slot on its upper side.
%
% veh is the numeric vehicle-parameter vector:
% veh(3) = wheelbase
% veh(4) = wheel tread
% veh(5) = front overhang
% veh(6) = rear overhang
% veh(7) = left overhang
% veh(8) = right overhang

persistent occ

%% Grid

res = 0.3;
W = 234;
H = 234;

origin_x = -(W/2)*res;
origin_y = -(H/2)*res;

%% Vehicle dimensions

wheelbase      = veh(3);
wheel_tread    = veh(4);
front_overhang = veh(5);
rear_overhang  = veh(6);
left_overhang  = veh(7);
right_overhang = veh(8);

car_len = front_overhang + wheelbase + rear_overhang;
car_wid = wheel_tread + left_overhang + right_overhang;

%% Parking-scene parameters

% Obstacle inflation, matching the costmap generator
expand = 0.5;

parked_car_len = car_len + expand;
parked_car_wid = car_wid + expand;

% Road boundaries
road_x_min = -14;
road_x_max =  14;
road_y_min = -2.2;
road_y_max =  2.2;

% Tight empty-slot length
% With the current ATOM dimensions, this gives about 0.4 m clearance
% at each end for the inflated ego footprint.
slot_extra_length = 2.0;%1.3
slot_length = car_len + slot_extra_length;
slot_center_x = 0;

% Parking strip beside the road
parking_strip_width = parked_car_wid + 0.6;
parking_y = road_y_max + parking_strip_width/2;
parking_y_max = road_y_max + parking_strip_width;

% Small separation between parked vehicles outside the empty slot
inter_car_gap = 0.3;

%% Generate the occupancy grid

if isempty(occ)

    [IX,IY] = meshgrid(0:W-1,0:H-1);

    X = origin_x + IX*res;
    Y = origin_y + IY*res;

    % Begin with the whole map occupied
    occ = ones(H,W);

    % Create the road and its parking strip
    free_x = [ ...
        road_x_min, road_x_max, ...
        road_x_max, road_x_min];

    free_y = [ ...
        road_y_min, road_y_min, ...
        parking_y_max, parking_y_max];

    occ(inpolygon(X,Y,free_x,free_y)) = 0;

    %% Parked-car positions

    % Distance from the slot centre to either adjacent car centre
    adjacent_offset = ...
        (slot_length + parked_car_len)/2;

    % Two cars on each side of the empty slot
    parked_car_x = [ ...
        -adjacent_offset - parked_car_len - inter_car_gap, ...
        -adjacent_offset, ...
         adjacent_offset, ...
         adjacent_offset + parked_car_len + inter_car_gap];

    %% Add the parked cars

    for k = 1:length(parked_car_x)

        car_x = parked_car_x(k);

        % The cars are parallel to the road:
        % length along x and width along y
        qx = [ ...
            -parked_car_len/2, ...
             parked_car_len/2, ...
             parked_car_len/2, ...
            -parked_car_len/2] + car_x;

        qy = [ ...
            -parked_car_wid/2, ...
            -parked_car_wid/2, ...
             parked_car_wid/2, ...
             parked_car_wid/2] + parking_y;

        occ(inpolygon(X,Y,qx,qy)) = 1;
    end
end

%% Starting pose

% Rear-axle centre, travelling east along the road
start_pose = [-10, 0, 0];%;%%;

%% Goal pose

% The parking slot is defined using its geometric centre, but Autoware's
% vehicle pose is the rear-axle centre.
body_center_from_rear_axle = ...
    (wheelbase + front_overhang - rear_overhang)/2;

goal_pose = [ ...
    slot_center_x - body_center_from_rear_axle, ...
    parking_y, ...
    0];

%% Costmap message

costmap.info.resolution = res;
costmap.info.width      = uint32(W);
costmap.info.height     = uint32(H);

costmap.info.origin.position.x = origin_x;
costmap.info.origin.position.y = origin_y;
costmap.info.origin.position.z = 0;

costmap.info.origin.orientation.x = 0;
costmap.info.origin.orientation.y = 0;
costmap.info.origin.orientation.z = 0;
costmap.info.origin.orientation.w = 1;

costmap.data = int8(occ*100);

end
